simulink model "car_control"  (R2026a)
settings: Solver=ode4  StopTime=80  FixedStep=0.01
values from neighbouring files (symbols this model uses):
  Af = 2    [control.m]
  Cd = 0.3    [control.m]
  g = 9.81    [control.m]
  Ki = m*wn^2    (= 1.8e-16)    [control.m]
  Kp = m*(2*zeta*wn - A)    (= 489.6)    [control.m]
  m = 2000    [control.m]
  mu = 0.005    [control.m]
  R = 15    [control.m]
  rho = 1.2    [control.m]
  uo = 0.5*rho*Cd*Af*xo^2 + m*g*sin(w) + mu*m*g*cos(w)    [control.m]
  w = 0.0599    [control.m]
  x0 = 0    [control.m]
  xo = 0.34    [control.m]
settings Model: Creator=stefa  LastModifiedBy=stefa

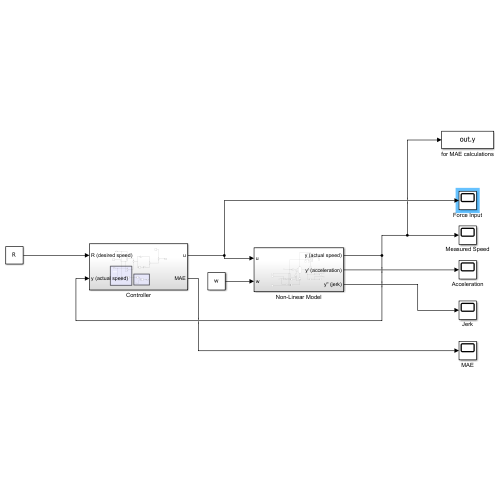
[thumbnail: Simulink's stored preview of the top-level diagram]
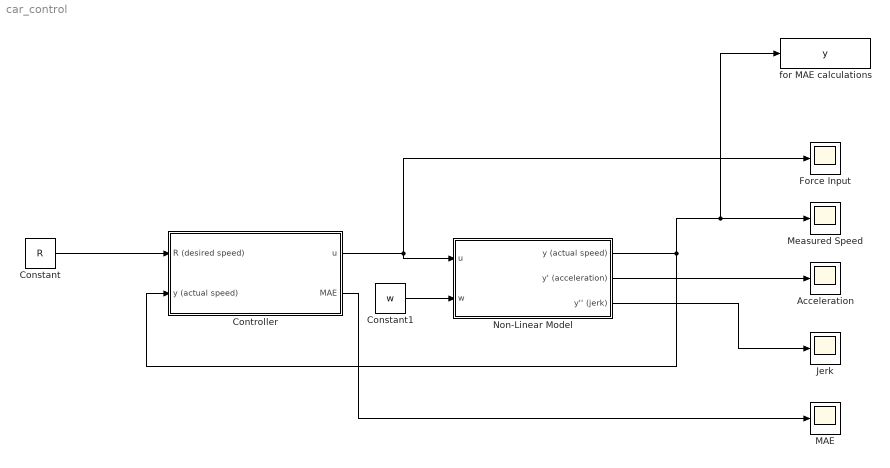
== system car_control ==
  Acceleration : Scope
      settings: ActiveDisplayYMinimum=-20.775756727567511  ActiveDisplayYMaximum=41.333021330885387  DataLoggingVariableName=ScopeData5
  Constant : Constant  Value=R
  Constant1 : Constant  Value=w
  Controller : Subsystem
  Force Input : Scope
      settings: ActiveDisplayYMinimum=2855.6527173902559  ActiveDisplayYMaximum=12310.41881216089  DataLoggingVariableName=ScopeData2
  Jerk : Scope
      settings: ActiveDisplayYMinimum=-3.6678846096277962  ActiveDisplayYMaximum=3.9531358038475974  DataLoggingVariableName=ScopeData6
  MAE : Scope
      settings: ActiveDisplayYMinimum=-12.547698677553527  ActiveDisplayYMaximum=18.821454719482258  DataLoggingVariableName=ScopeData7
  Measured Speed : Scope
      settings: ActiveDisplayYMinimum=-11.329486976749827  ActiveDisplayYMaximum=100.20895500102731
  Non-Linear Model : Subsystem
  for MAE calculations : ToWorkspace  VariableName=y  SaveFormat=Timeseries  SampleTime=-1
  wires:
  Controller/1(u) -> Non-Linear Model/1(u), Force Input/1
  Constant1/1 -> Non-Linear Model/2(w)
  Non-Linear Model/1(y (actual speed)) -> Controller/2(y (actual speed)), for MAE calculations/1, Measured Speed/1
  Constant/1 -> Controller/1(R (desired speed))
  Non-Linear Model/2(y' (acceleration)) -> Acceleration/1
  Non-Linear Model/3(y'' (jerk)) -> Jerk/1
  Controller/2(MAE) -> MAE/1

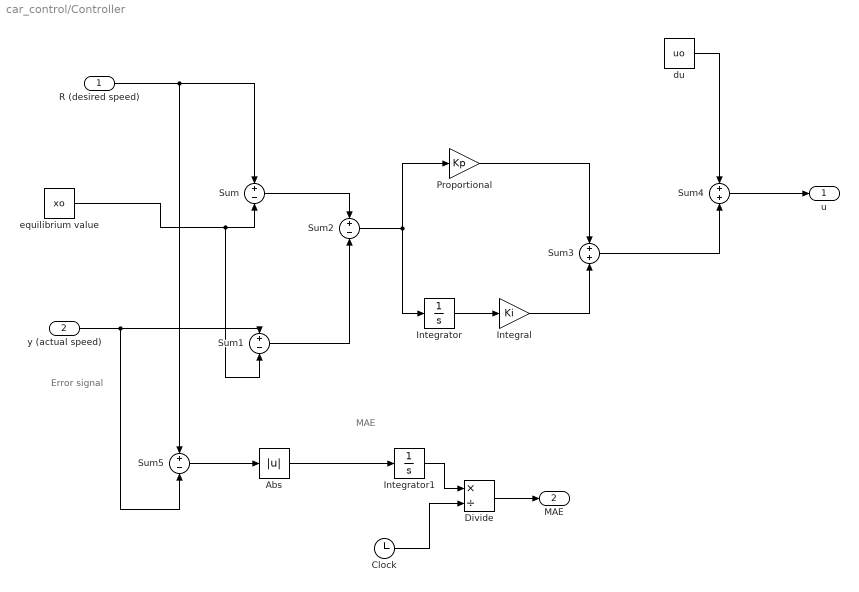
== system car_control/Controller ==
  note: MAE
  note: Error signal
  R (desired speed) : Inport
  y (actual speed) : Inport  Port=2
  Abs : Abs  SaturateOnIntegerOverflow=off
  Clock : Clock
  Divide : Product  Inputs=*/
  Integral : Gain  Gain=Ki
  Integrator : Integrator
  Integrator1 : Integrator
  Proportional : Gain  Gain=Kp
  Sum{,1..2,5} (4 alike) : Sum  Inputs=+-
  Sum3 : Sum
  Sum4 : Sum
  du : Constant  Value=uo
  equilibrium value : Constant  Value=xo
  u : Outport
  MAE : Outport  Port=2
  wires:
  R (desired speed)/1 -> Sum/1, Sum5/1
  equilibrium value/1 -> Sum/2, Sum1/2
  y (actual speed)/1 -> Sum1/1, Sum5/2
  Sum/1 -> Sum2/1
  Sum1/1 -> Sum2/2
  Sum2/1 -> Integrator/1, Proportional/1
  Integrator/1 -> Integral/1
  Proportional/1 -> Sum3/1
  Sum3/1 -> Sum4/2
  Sum4/1 -> u/1
  du/1 -> Sum4/1
  Integral/1 -> Sum3/2
  Sum5/1 -> Abs/1
  Abs/1 -> Integrator1/1
  Clock/1 -> Divide/2
  Integrator1/1 -> Divide/1
  Divide/1 -> MAE/1

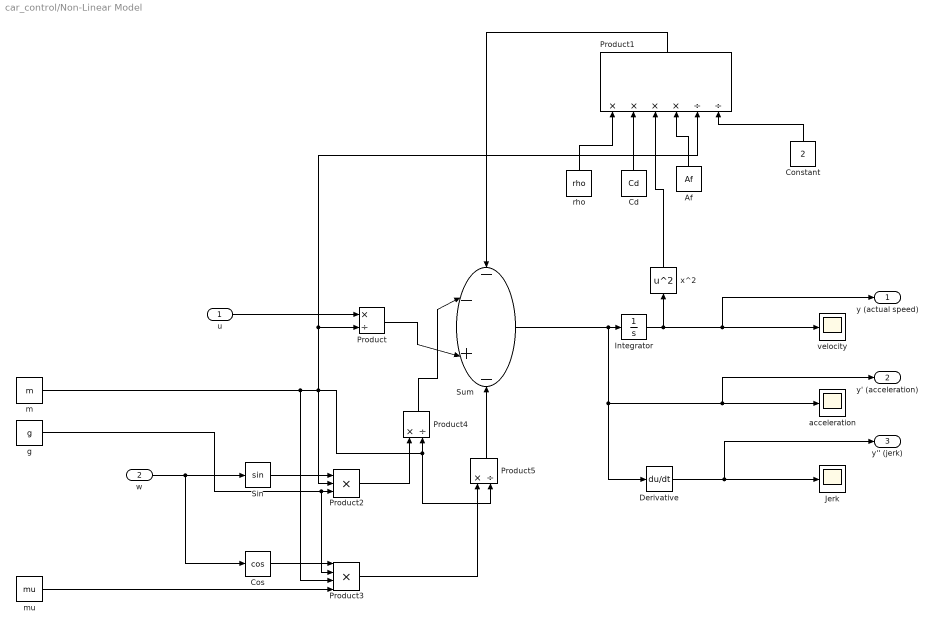
== system car_control/Non-Linear Model ==
  u : Inport
  w : Inport  Port=2
  Af : Constant  Value=Af
  Cd : Constant  Value=Cd
  Constant : Constant  Value=2
  Cos : Trigonometry  Operator=cos
  Derivative : Derivative
  Integrator : Integrator  InitialCondition=x0
  Jerk : Scope
      settings: ActiveDisplayYMinimum=-1.0725427232299787  ActiveDisplayYMaximum=2.8853427188943455  DataLoggingVariableName=ScopeData4
  Product : Product  Inputs=*/
  Product1 : Product  Inputs=****//
  Product2 : Product  Inputs=***
  Product3 : Product  Inputs=****
  Product4 : Product  Inputs=*/
  Product5 : Product  Inputs=*/
  Sin : Trigonometry
  Sum : Sum  Inputs=--+-
  acceleration : Scope
      settings: ActiveDisplayYMinimum=-1.6759629370118283  ActiveDisplayYMaximum=3.3754132792586082  DataLoggingVariableName=ScopeData3
  g : Constant  Value=g
  m : Constant  Value=m
  mu : Constant  Value=mu
  rho : Constant  Value=rho
  velocity : Scope
      settings: ActiveDisplayYMinimum=4.7924567222561487  ActiveDisplayYMaximum=20.307878770609037
  x^2 : Math  Operator=square
  y (actual speed) : Outport
  y' (acceleration) : Outport  Port=2
  y'' (jerk) : Outport  Port=3
  wires:
  m/1 -> Product5/2, Product4/2, Product2/2, Product/2, Product1/5, Product3/3
  u/1 -> Product/1
  Product/1 -> Sum/3
  Sum/1 -> y' (acceleration)/1, acceleration/1, Derivative/1, Integrator/1
  Integrator/1 -> x^2/1, y (actual speed)/1, velocity/1
  x^2/1 -> Product1/3
  Constant/1 -> Product1/6
  Af/1 -> Product1/4
  Cd/1 -> Product1/2
  rho/1 -> Product1/1
  Product1/1 -> Sum/1
  w/1 -> Sin/1, Cos/1
  Sin/1 -> Product2/1
  g/1 -> Product3/2, Product2/3
  Cos/1 -> Product3/1
  mu/1 -> Product3/4
  Product2/1 -> Product4/1
  Product4/1 -> Sum/2
  Product3/1 -> Product5/1
  Product5/1 -> Sum/4
  Derivative/1 -> Jerk/1, y'' (jerk)/1
